simulink model "rand_ramp"  (Simulink 4.00)
settings: Solver=ode45  StartTime=0.0  StopTime=100  RelTol=1e-3
settings Model: Creator=mcar  LastModifiedBy=mcar  BlockReductionOpt=off

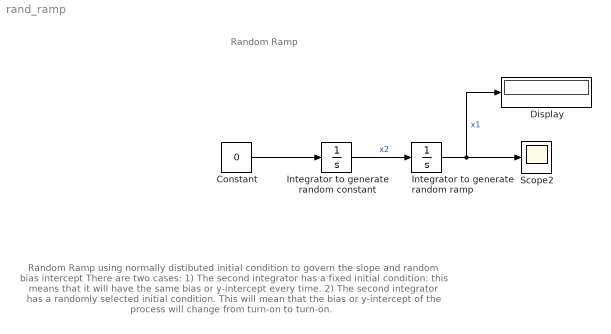
== system rand_ramp ==
  note: Random Ramp using normally distibuted initial condition
      | to govern the slope and random bias intercept
      | There are two cases:
      | 1) The second integrator has a fixed initial condition: this means that it
      | will have the same bias or y-intercept every time.
      | 2) The second integrator has a randomly selected initial condition.  This will
      | mean that the bias or y-intercept of the process will change from turn-on to turn-on.
  note: Random Ramp
  Constant : Constant  Value=0
  Display : Display
      settings: Format=short
  Integrator to generate random constant : Integrator  ExternalReset=none  InitialConditionSource=internal  InitialCondition=3+10*rand  LimitOutput=off  UpperSaturationLimit=inf  LowerSaturationLimit=-inf  ShowSaturationPort=off  ShowStatePort=off  AbsoluteTolerance=auto
  Integrator to generate random ramp : Integrator  ExternalReset=none  InitialConditionSource=internal  InitialCondition=300*rand  LimitOutput=off  UpperSaturationLimit=inf  LowerSaturationLimit=-inf  ShowSaturationPort=off  ShowStatePort=off  AbsoluteTolerance=auto
  Scope2 : Scope
      settings: TimeRange=100  YMin=0  YMax=1200  SaveToWorkspace=off  SaveName=ScopeData2  LimitDataPoints=on  MaxDataPoints=5000
  wires:
  Integrator to generate random constant/1 -> Integrator to generate random ramp/1  "x2"
  Integrator to generate random ramp/1 -> Scope2/1, Display/1  "x1"
  Constant/1 -> Integrator to generate random constant/1
